simulink model "Main_Simulation"  (R2025b)
settings: Solver=VariableStepAuto  StartTime=0.0  StopTime=10  RelTol=1e-3
settings Model: DataDictionary=DAB_Parameters.sldd  Creator=vivid  LastModifiedBy=vivid

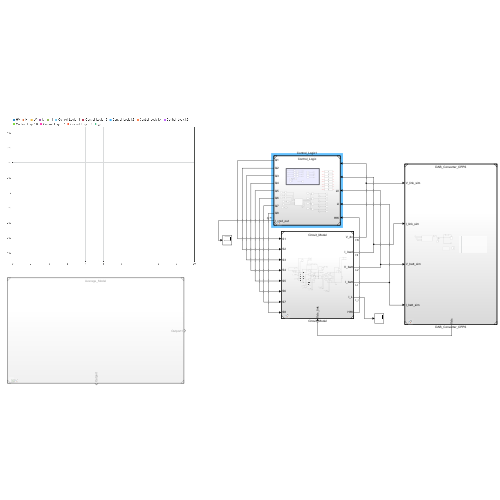
[thumbnail: Simulink's stored preview of the top-level diagram]
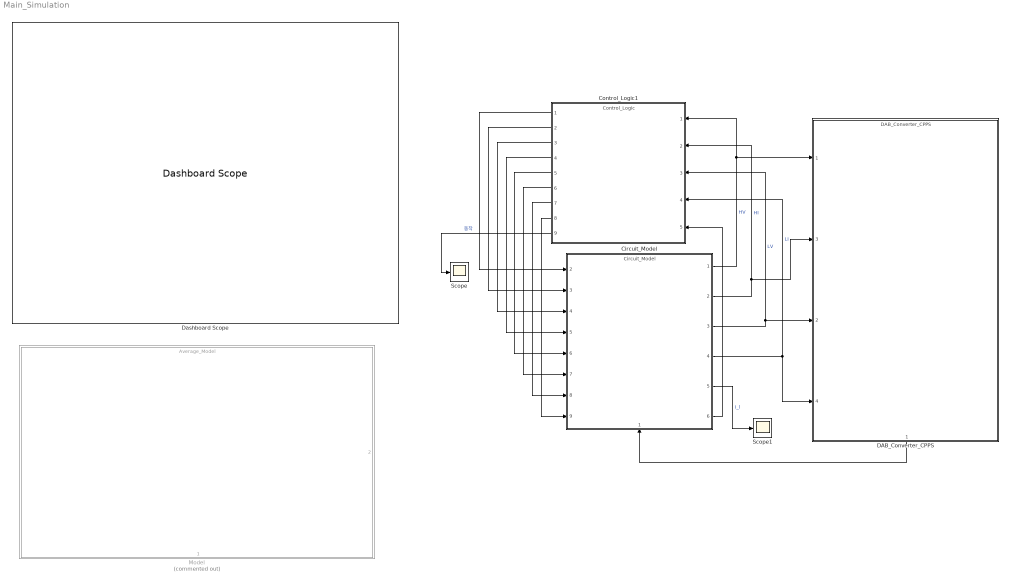
== system Main_Simulation ==
  Circuit_Model : ModelReference  ModelNameDialog=Circuit_Model.slx  SimulationMode=Normal  ModelReferenceVersion=1.15
      settings: PortSchema="{\"entries\":[{\"content\":{\"sides\":[{\"content\":{\"connectorIds\":[\"In2\",\"In3\",\"In4\",\"In5\",\"In6\",\"In7\",\"In8\",\"In9\"]},\"type\":\"ConnectorPlacement.EquallySpacedRectSide\",\"uuid\":\"38594a29-610e-4e16-ac58-80da3176b6ab\"},{\"content\":{\"connectorIds\":[\"Out1\",\"Out2\",\"Out3\",\"Out4\",\"Out5\",\"Out6\"],\"side\":\"RIGHT\"},\"type\":\"ConnectorPlacement.EquallySpacedRectSide\",\"uuid\":\"0547ad6e-86bd-4c8b-8c4c-506be515b270\"},{\"content\":{\"side\":\"TOP\"},\"type\":\"ConnectorPlacement.EquallySpacedRectSide\",\"uuid\":\"353d2b5d-724b-4234-a969-55b5ad94d399\"},{\"content\":{\"connectorIds\":[\"In1\"],\"side\":\"BOTTOM\"},\"type\":\"ConnectorPlacement.EquallySpacedRectSide\",\"uuid\":\"648c670a-bb52-4b09-9201-da27f824cf39\"}]},\"type\":\"ConnectorPlacement.EquallySpacedConnector\",\"uuid\":\"14d7ba85-855e-4ee6-9041-4db0cebf9bc5\"}],\"packageUris\":[\"http://schema.mathworks.com/mf0/Connector/R2020b\"],\"version\":\"1.0\"}"
  Control_Logic1 : ModelReference  ModelNameDialog=Control_Logic.slx  SimulationMode=Normal  ModelReferenceVersion=1.33
  DAB_Converter_CPPS : ModelReference  ModelNameDialog=DAB_Converter_CPPS.slx  SimulationMode=Normal  ModelReferenceVersion=1.13
      settings: PortSchema="{\"entries\":[{\"content\":{\"sides\":[{\"content\":{\"connectorIds\":[\"In4\",\"In2\",\"In3\",\"In1\"]},\"type\":\"ConnectorPlacement.EquallySpacedRectSide\",\"uuid\":\"7df16d4b-93d7-4b77-ae2b-1f752433f161\"},{\"content\":{\"side\":\"RIGHT\"},\"type\":\"ConnectorPlacement.EquallySpacedRectSide\",\"uuid\":\"2f928e84-a701-46fc-b504-55591f350ad6\"},{\"content\":{\"connectorIds\":[\"Out1\"],\"side\":\"TOP\"},\"type\":\"ConnectorPlacement.EquallySpacedRectSide\",\"uuid\":\"28d03347-600a-41f0-81cf-e688561cdbb0\"}]},\"type\":\"ConnectorPlacement.EquallySpacedConnector\",\"uuid\":\"c8cc4caa-e63b-4775-b150-2a5a2103dbf4\"}],\"packageUris\":[\"http://schema.mathworks.com/mf0/Connector/R2020b\"],\"version\":\"1.0\"}"
  Dashboard Scope : DashboardScope  FontColor=[0.0, 0.0, 0.0]
  Model : ModelReference  Commented=on  ModelNameDialog=Average_Model.slx  SimulationMode=Normal  ModelReferenceVersion=1.7
      settings: PortSchema="{\"entries\":[{\"content\":{\"sides\":[{\"content\":{},\"type\":\"ConnectorPlacement.EquallySpacedRectSide\",\"uuid\":\"07b0600c-ef2c-4839-989c-d4d13efdc1f5\"},{\"content\":{\"connectorIds\":[\"Out2\"],\"side\":\"RIGHT\"},\"type\":\"ConnectorPlacement.EquallySpacedRectSide\",\"uuid\":\"877db3d9-96a8-4aa9-a4b5-31a411037f9e\"},{\"content\":{\"side\":\"TOP\"},\"type\":\"ConnectorPlacement.EquallySpacedRectSide\",\"uuid\":\"eff5b5c5-338a-4f79-bb2e-95f622a9c199\"},{\"content\":{\"connectorIds\":[\"Out1\"],\"side\":\"BOTTOM\"},\"type\":\"ConnectorPlacement.EquallySpacedRectSide\",\"uuid\":\"660c2c95-0901-4e2c-9fd6-171e9e644d1d\"}]},\"type\":\"ConnectorPlacement.EquallySpacedConnector\",\"uuid\":\"03bc4459-e8ae-490b-a87f-f32195118c54\"}],\"packageUris\":[\"http://schema.mathworks.com/mf0/Connector/R2020b\"],\"version\":\"1.0\"}"
  Scope : Scope
  Scope1 : Scope
      settings: ActiveDisplayYMinimum=-2.0105199371046262E-11  ActiveDisplayYMaximum=1.9949020422365471E-11
  wires:
  DAB_Converter_CPPS/1 -> Circuit_Model/1
  Circuit_Model/1 -> DAB_Converter_CPPS/1, Control_Logic1/1  "HV"
  Circuit_Model/4 -> DAB_Converter_CPPS/4, Control_Logic1/4  "LI"
  Circuit_Model/2 -> Control_Logic1/2, DAB_Converter_CPPS/3  "HI"
  Circuit_Model/3 -> Control_Logic1/3, DAB_Converter_CPPS/2  "LV"
  Control_Logic1/1 -> Circuit_Model/2
  Control_Logic1/2 -> Circuit_Model/3
  Control_Logic1/3 -> Circuit_Model/4
  Control_Logic1/4 -> Circuit_Model/5
  Control_Logic1/5 -> Circuit_Model/6
  Control_Logic1/6 -> Circuit_Model/7
  Control_Logic1/7 -> Circuit_Model/8
  Control_Logic1/8 -> Circuit_Model/9
  Control_Logic1/9 -> Scope/1  "동작"
  Circuit_Model/5 -> Scope1/1  "I_l"
  Circuit_Model/6 -> Control_Logic1/5
